simulink library "sm_wheel_loader_lib"  (R2025a)
settings: Solver=VariableStepAuto  StartTime=0.0  StopTime=10.0  RelTol=1e-3
undefined symbols (not defined in the file): AToTOrificeVector, BiPOrificeVector, boomHEArea, boomREArea, BToTOrificeVector, fluids, GRake, GToothL, GToothR, HMPST, HydFcnParams, logLoad, Position, PToAOrificeVector, PToBOrificeVector, RakeL, RakeR, testInput, Wheel_Loader, X, Y, Z
libraries: sm_lib x694, fl_lib x183, nesl_utility x74, SimscapeFluids_lib x62, sdl_lib x25, cvt_components_lib x25, simulink_extras x5, $bdroot x4, wheel_loader_contact_lib x4, ee_lib x2, SignalEditorBlockLib x1, batteryecm_lib x1
(part 20 of 26)

== system sm_wheel_loader_lib/Wheel Loader Vehicle/Driveline/Driveline/Driveline 1D/Planetary RL/Ring Gear ==
  Bolts : sm_lib/Body Elements/File Solid  ExtGeomFileName=InWheelPlanetary_Ring_Bolts.STEP  UnitType=FromFile  ExtGeomFileUnits=m  StepReaderType=HEX  ExportConvexHullGeometry=off  InertiaType=Custom  BasedOnType=DensityFromFile  Density=1000  DensityUnits=kg/m^3  Mass=Wheel_Loader.bodyGroups(74).subGroups(2).inertialProperties.mass  MassUnits=kg  CenterOfMass=Wheel_Loader.bodyGroups(74).subGroups(2).inertialProperties.centerOfMass  CenterOfMassUnits=m  MomentsOfInertia=Wheel_Loader.bodyGroups(74).subGroups(2).inertialProperties.momentsOfInertia  MomentsOfInertiaUnits=kg*m^2  ProductsOfInertia=Wheel_Loader.bodyGroups(74).subGroups(2).inertialProperties.productsOfInertia  ProductsOfInertiaUnits=kg*m^2  GraphicType=FromGeometry  MarkerShape=Sphere  MarkerSize=10  GraphicVisPropType=SimpleVisualProperties  GraphicDiffuseColor=Wheel_Loader.bodyGroups(74).subGroups(2).visualProperties.rgb  GraphicOpacity=Wheel_Loader.bodyGroups(74).subGroups(2).visualProperties.opacity  GraphicSpecularColor=[0.5 0.5 0.5 1.0]  GraphicAmbientColor=[0.15 0.15 0.15 1.0]  GraphicEmissiveColor=[0.0 0.0 0.0 1.0]  GraphicShininess=75  DoExposeReferenceFrame=on  SerializedFrames=<Frames/>
  Ring : sm_lib/Body Elements/File Solid  ExtGeomFileName=InWheelPlanetary_Ring.STEP  UnitType=FromFile  ExtGeomFileUnits=m  StepReaderType=HEX  ExportConvexHullGeometry=off  InertiaType=Custom  BasedOnType=DensityFromFile  Density=1000  DensityUnits=kg/m^3  Mass=Wheel_Loader.bodyGroups(74).subGroups(1).inertialProperties.mass  MassUnits=kg  CenterOfMass=Wheel_Loader.bodyGroups(74).subGroups(1).inertialProperties.centerOfMass  CenterOfMassUnits=m  MomentsOfInertia=Wheel_Loader.bodyGroups(74).subGroups(1).inertialProperties.momentsOfInertia  MomentsOfInertiaUnits=kg*m^2  ProductsOfInertia=Wheel_Loader.bodyGroups(74).subGroups(1).inertialProperties.productsOfInertia  ProductsOfInertiaUnits=kg*m^2  GraphicType=FromGeometry  MarkerShape=Sphere  MarkerSize=10  GraphicVisPropType=SimpleVisualProperties  GraphicDiffuseColor=Wheel_Loader.bodyGroups(74).subGroups(1).visualProperties.rgb  GraphicOpacity=Wheel_Loader.bodyGroups(74).subGroups(1).visualProperties.opacity  GraphicSpecularColor=[0.5 0.5 0.5 1.0]  GraphicAmbientColor=[0.15 0.15 0.15 1.0]  GraphicEmissiveColor=[0.0 0.0 0.0 1.0]  GraphicShininess=75  DoExposeReferenceFrame=on  SerializedFrames=<Frames/>
  RingGear_Center : sm_lib/Frames and Transforms/Rigid Transform  RotationMethod=RotationMatrix  FollAlignAxisA=+X  BaseAlignAxisA=+Y  FollAlignAxisB=+Y  BaseAlignAxisB=+Z  RotationStandardAxis=+Z  RotationAngle=0.0  RotationAngleUnits=deg  RotationArbitraryAxis=[0 0 1]  RotationSequenceAxes=FollowerAxes  RotationSequence=XYX  RotationSequenceAngles=[0 0 0]  RotationSequenceAnglesUnits=deg  RotationMatrix=Wheel_Loader.coordSys(58).transform.rotation  Quaternion=[1 0 0 0]  TranslationMethod=Cartesian  TranslationCartesianOffset=Wheel_Loader.coordSys(58).transform.translation  TranslationCartesianOffsetUnits=m  TranslationStandardAxis=+Z  TranslationStandardOffset=0  TranslationStandardOffsetUnits=m  TranslationROffset=0  TranslationROffsetUnits=m  TranslationThetaOffset=0  TranslationThetaOffsetUnits=deg  TranslationZOffset=0  TranslationZOffsetUnits=m
  B : PMIOPort  Side=Left
  connections:
  RingGear_Center/RConn1 -- B/RConn1
  Bolts/RConn1 -- RingGear_Center/LConn1 -- Ring/RConn1

== system sm_wheel_loader_lib/Wheel Loader Vehicle/Driveline/Driveline/Driveline 1D/Planetary RR/Carrier ==
  Bolts : sm_lib/Body Elements/File Solid  ExtGeomFileName=InWheelPlanetary_Carrier_Bolts.STEP  UnitType=FromFile  ExtGeomFileUnits=m  StepReaderType=HEX  ExportConvexHullGeometry=off  InertiaType=Custom  BasedOnType=DensityFromFile  Density=1000  DensityUnits=kg/m^3  Mass=Wheel_Loader.bodyGroups(75).subGroups(2).inertialProperties.mass  MassUnits=kg  CenterOfMass="Wheel_Loader.bodyGroups(75).subGroups(2).inertialProperties.centerOfMass-[0 0.000000601963208   0.000000302490290]'"  CenterOfMassUnits=m  MomentsOfInertia=Wheel_Loader.bodyGroups(75).subGroups(2).inertialProperties.momentsOfInertia  MomentsOfInertiaUnits=kg*m^2  ProductsOfInertia=Wheel_Loader.bodyGroups(75).subGroups(2).inertialProperties.productsOfInertia  ProductsOfInertiaUnits=kg*m^2  GraphicType=FromGeometry  MarkerShape=Sphere  MarkerSize=10  GraphicVisPropType=SimpleVisualProperties  GraphicDiffuseColor=Wheel_Loader.bodyGroups(75).subGroups(2).visualProperties.rgb  GraphicOpacity=casing_opc  GraphicSpecularColor=[0.5 0.5 0.5 1.0]  GraphicAmbientColor=[0.15 0.15 0.15 1.0]  GraphicEmissiveColor=[0.0 0.0 0.0 1.0]  GraphicShininess=75  DoExposeReferenceFrame=on  SerializedFrames=<Frames/>
  Carrier : sm_lib/Body Elements/File Solid  ExtGeomFileName=InWheelPlanetary_Carrier.STEP  UnitType=FromFile  ExtGeomFileUnits=m  StepReaderType=HEX  ExportConvexHullGeometry=off  InertiaType=Custom  BasedOnType=DensityFromFile  Density=1000  DensityUnits=kg/m^3  Mass=Wheel_Loader.bodyGroups(75).subGroups(1).inertialProperties.mass  MassUnits=kg  CenterOfMass="Wheel_Loader.bodyGroups(75).subGroups(1).inertialProperties.centerOfMass-[0 -0.000000000960056  -0.000000002279457]'"  CenterOfMassUnits=m  MomentsOfInertia=Wheel_Loader.bodyGroups(75).subGroups(1).inertialProperties.momentsOfInertia  MomentsOfInertiaUnits=kg*m^2  ProductsOfInertia=Wheel_Loader.bodyGroups(75).subGroups(1).inertialProperties.productsOfInertia  ProductsOfInertiaUnits=kg*m^2  GraphicType=FromGeometry  MarkerShape=Sphere  MarkerSize=10  GraphicVisPropType=SimpleVisualProperties  GraphicDiffuseColor=Wheel_Loader.bodyGroups(75).subGroups(1).visualProperties.rgb  GraphicOpacity=casing_opc  GraphicSpecularColor=[0.5 0.5 0.5 1.0]  GraphicAmbientColor=[0.15 0.15 0.15 1.0]  GraphicEmissiveColor=[0.0 0.0 0.0 1.0]  GraphicShininess=75  DoExposeReferenceFrame=on  SerializedFrames=<Frames/>
  RT1_Carrier_Planet1 : sm_lib/Frames and Transforms/Rigid Transform  RotationMethod=StandardAxis  FollAlignAxisA=+X  BaseAlignAxisA=+Y  FollAlignAxisB=+Y  BaseAlignAxisB=+Z  RotationStandardAxis=+Z  RotationAngle=3.5  RotationAngleUnits=deg  RotationArbitraryAxis=[0 0 1]  RotationSequenceAxes=FollowerAxes  RotationSequence=XYX  RotationSequenceAngles=[0 0 0]  RotationSequenceAnglesUnits=deg  RotationMatrix=Wheel_Loader.coordSys(58).transform.rotation  Quaternion=[1 0 0 0]  TranslationMethod=None  TranslationCartesianOffset=Wheel_Loader.coordSys(58).transform.translation  TranslationCartesianOffsetUnits=m  TranslationStandardAxis=+X  TranslationStandardOffset=-0.037861875000022  TranslationStandardOffsetUnits=m  TranslationROffset=0  TranslationROffsetUnits=m  TranslationThetaOffset=0  TranslationThetaOffsetUnits=deg  TranslationZOffset=0  TranslationZOffsetUnits=m
  RT1_Carrier_Planet2 : sm_lib/Frames and Transforms/Rigid Transform  RotationMethod=StandardAxis  FollAlignAxisA=+X  BaseAlignAxisA=+Y  FollAlignAxisB=+Y  BaseAlignAxisB=+Z  RotationStandardAxis=+Z  RotationAngle=3.5+120  RotationAngleUnits=deg  RotationArbitraryAxis=[0 0 1]  RotationSequenceAxes=FollowerAxes  RotationSequence=XYX  RotationSequenceAngles=[0 0 0]  RotationSequenceAnglesUnits=deg  RotationMatrix=Wheel_Loader.coordSys(58).transform.rotation  Quaternion=[1 0 0 0]  TranslationMethod=None  TranslationCartesianOffset=Wheel_Loader.coordSys(58).transform.translation  TranslationCartesianOffsetUnits=m  TranslationStandardAxis=+X  TranslationStandardOffset=-0.037861875000022  TranslationStandardOffsetUnits=m  TranslationROffset=0  TranslationROffsetUnits=m  TranslationThetaOffset=0  TranslationThetaOffsetUnits=deg  TranslationZOffset=0  TranslationZOffsetUnits=m
  RT1_Carrier_Planet3 : sm_lib/Frames and Transforms/Rigid Transform  RotationMethod=StandardAxis  FollAlignAxisA=+X  BaseAlignAxisA=+Y  FollAlignAxisB=+Y  BaseAlignAxisB=+Z  RotationStandardAxis=+Z  RotationAngle=3.5+240  RotationAngleUnits=deg  RotationArbitraryAxis=[0 0 1]  RotationSequenceAxes=FollowerAxes  RotationSequence=XYX  RotationSequenceAngles=[0 0 0]  RotationSequenceAnglesUnits=deg  RotationMatrix=Wheel_Loader.coordSys(58).transform.rotation  Quaternion=[1 0 0 0]  TranslationMethod=None  TranslationCartesianOffset=Wheel_Loader.coordSys(58).transform.translation  TranslationCartesianOffsetUnits=m  TranslationStandardAxis=+X  TranslationStandardOffset=-0.037861875000022  TranslationStandardOffsetUnits=m  TranslationROffset=0  TranslationROffsetUnits=m  TranslationThetaOffset=0  TranslationThetaOffsetUnits=deg  TranslationZOffset=0  TranslationZOffsetUnits=m
  RT2_Carrier_Planet1 : sm_lib/Frames and Transforms/Rigid Transform  RotationMethod=StandardAxis  FollAlignAxisA=+X  BaseAlignAxisA=+Y  FollAlignAxisB=+Y  BaseAlignAxisB=+Z  RotationStandardAxis=+Z  RotationAngle=-3.5  RotationAngleUnits=deg  RotationArbitraryAxis=[0 0 1]  RotationSequenceAxes=FollowerAxes  RotationSequence=XYX  RotationSequenceAngles=[0 0 0]  RotationSequenceAnglesUnits=deg  RotationMatrix=Wheel_Loader.coordSys(58).transform.rotation  Quaternion=[1 0 0 0]  TranslationMethod=StandardAxis  TranslationCartesianOffset=Wheel_Loader.coordSys(58).transform.translation  TranslationCartesianOffsetUnits=m  TranslationStandardAxis=+X  TranslationStandardOffset=-0.0378618750  TranslationStandardOffsetUnits=m  TranslationROffset=0  TranslationROffsetUnits=m  TranslationThetaOffset=0  TranslationThetaOffsetUnits=deg  TranslationZOffset=0  TranslationZOffsetUnits=m
  RT2_Carrier_Planet2 : sm_lib/Frames and Transforms/Rigid Transform  RotationMethod=StandardAxis  FollAlignAxisA=+X  BaseAlignAxisA=+Y  FollAlignAxisB=+Y  BaseAlignAxisB=+Z  RotationStandardAxis=+Z  RotationAngle=-3.5  RotationAngleUnits=deg  RotationArbitraryAxis=[0 0 1]  RotationSequenceAxes=FollowerAxes  RotationSequence=XYX  RotationSequenceAngles=[0 0 0]  RotationSequenceAnglesUnits=deg  RotationMatrix=Wheel_Loader.coordSys(58).transform.rotation  Quaternion=[1 0 0 0]  TranslationMethod=StandardAxis  TranslationCartesianOffset=Wheel_Loader.coordSys(58).transform.translation  TranslationCartesianOffsetUnits=m  TranslationStandardAxis=+X  TranslationStandardOffset=-0.0378618750  TranslationStandardOffsetUnits=m  TranslationROffset=0  TranslationROffsetUnits=m  TranslationThetaOffset=0  TranslationThetaOffsetUnits=deg  TranslationZOffset=0  TranslationZOffsetUnits=m
  RT2_Carrier_Planet3 : sm_lib/Frames and Transforms/Rigid Transform  RotationMethod=StandardAxis  FollAlignAxisA=+X  BaseAlignAxisA=+Y  FollAlignAxisB=+Y  BaseAlignAxisB=+Z  RotationStandardAxis=+Z  RotationAngle=-3.5  RotationAngleUnits=deg  RotationArbitraryAxis=[0 0 1]  RotationSequenceAxes=FollowerAxes  RotationSequence=XYX  RotationSequenceAngles=[0 0 0]  RotationSequenceAnglesUnits=deg  RotationMatrix=Wheel_Loader.coordSys(58).transform.rotation  Quaternion=[1 0 0 0]  TranslationMethod=StandardAxis  TranslationCartesianOffset=Wheel_Loader.coordSys(58).transform.translation  TranslationCartesianOffsetUnits=m  TranslationStandardAxis=+X  TranslationStandardOffset=-0.0378618750  TranslationStandardOffsetUnits=m  TranslationROffset=0  TranslationROffsetUnits=m  TranslationThetaOffset=0  TranslationThetaOffsetUnits=deg  TranslationZOffset=0  TranslationZOffsetUnits=m
  RT_RearAxle_Carrier : sm_lib/Frames and Transforms/Rigid Transform  RotationMethod=RotationMatrix  FollAlignAxisA=+X  BaseAlignAxisA=+Y  FollAlignAxisB=+Y  BaseAlignAxisB=+Z  RotationStandardAxis=+Z  RotationAngle=0.0  RotationAngleUnits=deg  RotationArbitraryAxis=[0 0 1]  RotationSequenceAxes=FollowerAxes  RotationSequence=XYX  RotationSequenceAngles=[0 0 0]  RotationSequenceAnglesUnits=deg  RotationMatrix=Wheel_Loader.coordSys(58).transform.rotation  Quaternion=[1 0 0 0]  TranslationMethod=Cartesian  TranslationCartesianOffset=Wheel_Loader.coordSys(58).transform.translation  TranslationCartesianOffsetUnits=m  TranslationStandardAxis=+Z  TranslationStandardOffset=0  TranslationStandardOffsetUnits=m  TranslationROffset=0  TranslationROffsetUnits=m  TranslationThetaOffset=0  TranslationThetaOffsetUnits=deg  TranslationZOffset=0  TranslationZOffsetUnits=m
  B : PMIOPort  Side=Left
  F1 : PMIOPort  Port=2  Side=Right
  F2 : PMIOPort  Port=3  Side=Right
  F3 : PMIOPort  Port=4  Side=Right
  connections:
  F3/RConn1 -- RT2_Carrier_Planet3/RConn1
  RT2_Carrier_Planet3/LConn1 -- RT1_Carrier_Planet3/RConn1
  RT2_Carrier_Planet2/LConn1 -- RT1_Carrier_Planet2/RConn1
  F2/RConn1 -- RT2_Carrier_Planet2/RConn1
  Carrier/RConn1 -- RT_RearAxle_Carrier/LConn1 -- Bolts/RConn1
  RT1_Carrier_Planet3/LConn1 -- RT1_Carrier_Planet2/LConn1 -- RT1_Carrier_Planet1/LConn1 -- RT_RearAxle_Carrier/RConn1 -- B/RConn1
  F1/RConn1 -- RT2_Carrier_Planet1/RConn1
  RT2_Carrier_Planet1/LConn1 -- RT1_Carrier_Planet1/RConn1

== system sm_wheel_loader_lib/Wheel Loader Vehicle/Driveline/Driveline/Driveline 1D/Planetary RR/Ring Gear ==
  Bolts : sm_lib/Body Elements/File Solid  ExtGeomFileName=InWheelPlanetary_Ring_Bolts.STEP  UnitType=FromFile  ExtGeomFileUnits=m  StepReaderType=HEX  ExportConvexHullGeometry=off  InertiaType=Custom  BasedOnType=DensityFromFile  Density=1000  DensityUnits=kg/m^3  Mass=Wheel_Loader.bodyGroups(74).subGroups(2).inertialProperties.mass  MassUnits=kg  CenterOfMass=Wheel_Loader.bodyGroups(74).subGroups(2).inertialProperties.centerOfMass  CenterOfMassUnits=m  MomentsOfInertia=Wheel_Loader.bodyGroups(74).subGroups(2).inertialProperties.momentsOfInertia  MomentsOfInertiaUnits=kg*m^2  ProductsOfInertia=Wheel_Loader.bodyGroups(74).subGroups(2).inertialProperties.productsOfInertia  ProductsOfInertiaUnits=kg*m^2  GraphicType=FromGeometry  MarkerShape=Sphere  MarkerSize=10  GraphicVisPropType=SimpleVisualProperties  GraphicDiffuseColor=Wheel_Loader.bodyGroups(74).subGroups(2).visualProperties.rgb  GraphicOpacity=Wheel_Loader.bodyGroups(74).subGroups(2).visualProperties.opacity  GraphicSpecularColor=[0.5 0.5 0.5 1.0]  GraphicAmbientColor=[0.15 0.15 0.15 1.0]  GraphicEmissiveColor=[0.0 0.0 0.0 1.0]  GraphicShininess=75  DoExposeReferenceFrame=on  SerializedFrames=<Frames/>
  Ring : sm_lib/Body Elements/File Solid  ExtGeomFileName=InWheelPlanetary_Ring.STEP  UnitType=FromFile  ExtGeomFileUnits=m  StepReaderType=HEX  ExportConvexHullGeometry=off  InertiaType=Custom  BasedOnType=DensityFromFile  Density=1000  DensityUnits=kg/m^3  Mass=Wheel_Loader.bodyGroups(74).subGroups(1).inertialProperties.mass  MassUnits=kg  CenterOfMass=Wheel_Loader.bodyGroups(74).subGroups(1).inertialProperties.centerOfMass  CenterOfMassUnits=m  MomentsOfInertia=Wheel_Loader.bodyGroups(74).subGroups(1).inertialProperties.momentsOfInertia  MomentsOfInertiaUnits=kg*m^2  ProductsOfInertia=Wheel_Loader.bodyGroups(74).subGroups(1).inertialProperties.productsOfInertia  ProductsOfInertiaUnits=kg*m^2  GraphicType=FromGeometry  MarkerShape=Sphere  MarkerSize=10  GraphicVisPropType=SimpleVisualProperties  GraphicDiffuseColor=Wheel_Loader.bodyGroups(74).subGroups(1).visualProperties.rgb  GraphicOpacity=Wheel_Loader.bodyGroups(74).subGroups(1).visualProperties.opacity  GraphicSpecularColor=[0.5 0.5 0.5 1.0]  GraphicAmbientColor=[0.15 0.15 0.15 1.0]  GraphicEmissiveColor=[0.0 0.0 0.0 1.0]  GraphicShininess=75  DoExposeReferenceFrame=on  SerializedFrames=<Frames/>
  RingGear_Center : sm_lib/Frames and Transforms/Rigid Transform  RotationMethod=RotationMatrix  FollAlignAxisA=+X  BaseAlignAxisA=+Y  FollAlignAxisB=+Y  BaseAlignAxisB=+Z  RotationStandardAxis=+Z  RotationAngle=0.0  RotationAngleUnits=deg  RotationArbitraryAxis=[0 0 1]  RotationSequenceAxes=FollowerAxes  RotationSequence=XYX  RotationSequenceAngles=[0 0 0]  RotationSequenceAnglesUnits=deg  RotationMatrix=Wheel_Loader.coordSys(58).transform.rotation  Quaternion=[1 0 0 0]  TranslationMethod=Cartesian  TranslationCartesianOffset=Wheel_Loader.coordSys(58).transform.translation  TranslationCartesianOffsetUnits=m  TranslationStandardAxis=+Z  TranslationStandardOffset=0  TranslationStandardOffsetUnits=m  TranslationROffset=0  TranslationROffsetUnits=m  TranslationThetaOffset=0  TranslationThetaOffsetUnits=deg  TranslationZOffset=0  TranslationZOffsetUnits=m
  B : PMIOPort  Side=Left
  connections:
  Ring/RConn1 -- RingGear_Center/LConn1 -- Bolts/RConn1
  RingGear_Center/RConn1 -- B/RConn1

== system sm_wheel_loader_lib/Wheel Loader Vehicle/Driveline/Driveline/Driveline 3D/Center Shaft/Center Bearing ==
  Center_Bearing : sm_lib/Body Elements/File Solid  ExtGeomFileName=Driveline_Center_Bearing.STEP  UnitType=FromFile  ExtGeomFileUnits=m  StepReaderType=HEX  ExportConvexHullGeometry=off  InertiaType=Custom  BasedOnType=DensityFromFile  Density=1000  DensityUnits=kg/m^3  Mass=Wheel_Loader.bodyGroups(41).subGroups(1).inertialProperties.mass  MassUnits=kg  CenterOfMass=Wheel_Loader.bodyGroups(41).subGroups(1).inertialProperties.centerOfMass  CenterOfMassUnits=m  MomentsOfInertia=Wheel_Loader.bodyGroups(41).subGroups(1).inertialProperties.momentsOfInertia  MomentsOfInertiaUnits=kg*m^2  ProductsOfInertia=Wheel_Loader.bodyGroups(41).subGroups(1).inertialProperties.productsOfInertia  ProductsOfInertiaUnits=kg*m^2  GraphicType=FromGeometry  MarkerShape=Sphere  MarkerSize=10  GraphicVisPropType=SimpleVisualProperties  GraphicDiffuseColor=Wheel_Loader.bodyGroups(41).subGroups(1).visualProperties.rgb  GraphicOpacity=Wheel_Loader.bodyGroups(41).subGroups(1).visualProperties.opacity  GraphicSpecularColor=[0.5 0.5 0.5 1.0]  GraphicAmbientColor=[0.15 0.15 0.15 1.0]  GraphicEmissiveColor=[0.0 0.0 0.0 1.0]  GraphicShininess=75  DoExposeReferenceFrame=on  SerializedFrames=<Frames/>
  RT_MidShipShaft_CentreBearingDriveShaft : sm_lib/Frames and Transforms/Rigid Transform  RotationMethod=RotationMatrix  FollAlignAxisA=+X  BaseAlignAxisA=+Y  FollAlignAxisB=+Y  BaseAlignAxisB=+Z  RotationStandardAxis=+Z  RotationAngle=0.0  RotationAngleUnits=deg  RotationArbitraryAxis=[0 0 1]  RotationSequenceAxes=FollowerAxes  RotationSequence=XYX  RotationSequenceAngles=[0 0 0]  RotationSequenceAnglesUnits=deg  RotationMatrix=Wheel_Loader.coordSys(22).transform.rotation  Quaternion=[1 0 0 0]  TranslationMethod=Cartesian  TranslationCartesianOffset=Wheel_Loader.coordSys(22).transform.translation  TranslationCartesianOffsetUnits=m  TranslationStandardAxis=+Z  TranslationStandardOffset=0  TranslationStandardOffsetUnits=m  TranslationROffset=0  TranslationROffsetUnits=m  TranslationThetaOffset=0  TranslationThetaOffsetUnits=deg  TranslationZOffset=0  TranslationZOffsetUnits=m
  RT_RearDriveShaft_CenterBearingDriveShaft : sm_lib/Frames and Transforms/Rigid Transform  RotationMethod=RotationMatrix  FollAlignAxisA=+X  BaseAlignAxisA=+Y  FollAlignAxisB=+Y  BaseAlignAxisB=+Z  RotationStandardAxis=+Z  RotationAngle=0.0  RotationAngleUnits=deg  RotationArbitraryAxis=[0 0 1]  RotationSequenceAxes=FollowerAxes  RotationSequence=XYX  RotationSequenceAngles=[0 0 0]  RotationSequenceAnglesUnits=deg  RotationMatrix=Wheel_Loader.coordSys(22).transform.rotation  Quaternion=[1 0 0 0]  TranslationMethod=Cartesian  TranslationCartesianOffset=Wheel_Loader.coordSys(22).transform.translation  TranslationCartesianOffsetUnits=m  TranslationStandardAxis=+Z  TranslationStandardOffset=0  TranslationStandardOffsetUnits=m  TranslationROffset=0  TranslationROffsetUnits=m  TranslationThetaOffset=0  TranslationThetaOffsetUnits=deg  TranslationZOffset=0  TranslationZOffsetUnits=m
  B1 : PMIOPort  Side=Left
  B2 : PMIOPort  Port=2  Side=Right
  connections:
  RT_RearDriveShaft_CenterBearingDriveShaft/RConn1 -- B2/RConn1
  RT_MidShipShaft_CentreBearingDriveShaft/RConn1 -- B1/RConn1
  Center_Bearing/RConn1 -- RT_MidShipShaft_CentreBearingDriveShaft/LConn1 -- RT_RearDriveShaft_CenterBearingDriveShaft/LConn1

== system sm_wheel_loader_lib/Wheel Loader Vehicle/Driveline/Driveline/Driveline 3D/Center Shaft/Shaft Midship ==
  Intermediate_Shaft_Midship : sm_lib/Body Elements/File Solid  ExtGeomFileName=Driveline_Intermediate_Shaft_Midship.STEP  UnitType=FromFile  ExtGeomFileUnits=m  StepReaderType=HEX  ExportConvexHullGeometry=off  InertiaType=Custom  BasedOnType=DensityFromFile  Density=1000  DensityUnits=kg/m^3  Mass=Wheel_Loader.bodyGroups(40).subGroups(1).inertialProperties.mass  MassUnits=kg  CenterOfMass=Wheel_Loader.bodyGroups(40).subGroups(1).inertialProperties.centerOfMass  CenterOfMassUnits=m  MomentsOfInertia=Wheel_Loader.bodyGroups(40).subGroups(1).inertialProperties.momentsOfInertia  MomentsOfInertiaUnits=kg*m^2  ProductsOfInertia=Wheel_Loader.bodyGroups(40).subGroups(1).inertialProperties.productsOfInertia  ProductsOfInertiaUnits=kg*m^2  GraphicType=FromGeometry  MarkerShape=Sphere  MarkerSize=10  GraphicVisPropType=SimpleVisualProperties  GraphicDiffuseColor=Wheel_Loader.bodyGroups(40).subGroups(1).visualProperties.rgb  GraphicOpacity=Wheel_Loader.bodyGroups(40).subGroups(1).visualProperties.opacity  GraphicSpecularColor=[0.5 0.5 0.5 1.0]  GraphicAmbientColor=[0.15 0.15 0.15 1.0]  GraphicEmissiveColor=[0.0 0.0 0.0 1.0]  GraphicShininess=75  DoExposeReferenceFrame=on  SerializedFrames=<Frames/>
  RT_FrontDriveShaft_MidShipShaft : sm_lib/Frames and Transforms/Rigid Transform  RotationMethod=RotationMatrix  FollAlignAxisA=+X  BaseAlignAxisA=+Y  FollAlignAxisB=+Y  BaseAlignAxisB=+Z  RotationStandardAxis=+Z  RotationAngle=0.0  RotationAngleUnits=deg  RotationArbitraryAxis=[0 0 1]  RotationSequenceAxes=FollowerAxes  RotationSequence=XYX  RotationSequenceAngles=[0 0 0]  RotationSequenceAnglesUnits=deg  RotationMatrix=Wheel_Loader.coordSys(22).transform.rotation  Quaternion=[1 0 0 0]  TranslationMethod=Cartesian  TranslationCartesianOffset=Wheel_Loader.coordSys(22).transform.translation  TranslationCartesianOffsetUnits=m  TranslationStandardAxis=+Z  TranslationStandardOffset=0  TranslationStandardOffsetUnits=m  TranslationROffset=0  TranslationROffsetUnits=m  TranslationThetaOffset=0  TranslationThetaOffsetUnits=deg  TranslationZOffset=0  TranslationZOffsetUnits=m
  B1 : PMIOPort  Side=Left
  F1 : PMIOPort  Port=2  Side=Right
  connections:
  F1/RConn1 -- RT_FrontDriveShaft_MidShipShaft/RConn1 -- B1/RConn1
  Intermediate_Shaft_Midship/RConn1 -- RT_FrontDriveShaft_MidShipShaft/LConn1

== system sm_wheel_loader_lib/Wheel Loader Vehicle/Driveline/Driveline/Driveline 3D/Differential F/Ring Gear ==
  Casing_A : sm_lib/Body Elements/File Solid  ExtGeomFileName=DiffF_Casing_A.STEP  UnitType=FromFile  ExtGeomFileUnits=m  StepReaderType=HEX  ExportConvexHullGeometry=off  InertiaType=Custom  BasedOnType=DensityFromFile  Density=1000  DensityUnits=kg/m^3  Mass=Wheel_Loader.bodyGroups(68).subGroups(1).inertialProperties.mass  MassUnits=kg  CenterOfMass=Wheel_Loader.bodyGroups(68).subGroups(1).inertialProperties.centerOfMass  CenterOfMassUnits=m  MomentsOfInertia=Wheel_Loader.bodyGroups(68).subGroups(1).inertialProperties.momentsOfInertia  MomentsOfInertiaUnits=kg*m^2  ProductsOfInertia=Wheel_Loader.bodyGroups(68).subGroups(1).inertialProperties.productsOfInertia  ProductsOfInertiaUnits=kg*m^2  GraphicType=FromGeometry  MarkerShape=Sphere  MarkerSize=10  GraphicVisPropType=SimpleVisualProperties  GraphicDiffuseColor=Wheel_Loader.bodyGroups(68).subGroups(1).visualProperties.rgb  GraphicOpacity=diff_casing_opc  GraphicSpecularColor=[0.5 0.5 0.5 1.0]  GraphicAmbientColor=[0.15 0.15 0.15 1.0]  GraphicEmissiveColor=[0.0 0.0 0.0 1.0]  GraphicShininess=75  DoExposeReferenceFrame=on  SerializedFrames=<Frames/>
  Casing_B : sm_lib/Body Elements/File Solid  ExtGeomFileName=DiffF_Casing_B.STEP  UnitType=FromFile  ExtGeomFileUnits=m  StepReaderType=HEX  ExportConvexHullGeometry=off  InertiaType=Custom  BasedOnType=DensityFromFile  Density=1000  DensityUnits=kg/m^3  Mass=Wheel_Loader.bodyGroups(68).subGroups(2).inertialProperties.mass  MassUnits=kg  CenterOfMass=Wheel_Loader.bodyGroups(68).subGroups(2).inertialProperties.centerOfMass  CenterOfMassUnits=m  MomentsOfInertia=Wheel_Loader.bodyGroups(68).subGroups(2).inertialProperties.momentsOfInertia  MomentsOfInertiaUnits=kg*m^2  ProductsOfInertia=Wheel_Loader.bodyGroups(68).subGroups(2).inertialProperties.productsOfInertia  ProductsOfInertiaUnits=kg*m^2  GraphicType=FromGeometry  MarkerShape=Sphere  MarkerSize=10  GraphicVisPropType=SimpleVisualProperties  GraphicDiffuseColor=Wheel_Loader.bodyGroups(68).subGroups(2).visualProperties.rgb  GraphicOpacity=diff_casing_opc  GraphicSpecularColor=[0.5 0.5 0.5 1.0]  GraphicAmbientColor=[0.15 0.15 0.15 1.0]  GraphicEmissiveColor=[0.0 0.0 0.0 1.0]  GraphicShininess=75  DoExposeReferenceFrame=on  SerializedFrames=<Frames/>
  RT_FDL_StubShaft_RingGear : sm_lib/Frames and Transforms/Rigid Transform  RotationMethod=RotationMatrix  FollAlignAxisA=+X  BaseAlignAxisA=+Y  FollAlignAxisB=+Y  BaseAlignAxisB=+Z  RotationStandardAxis=+Z  RotationAngle=0.0  RotationAngleUnits=deg  RotationArbitraryAxis=[0 0 1]  RotationSequenceAxes=FollowerAxes  RotationSequence=XYX  RotationSequenceAngles=[0 0 0]  RotationSequenceAnglesUnits=deg  RotationMatrix=Wheel_Loader.coordSys(43).transform.rotation  Quaternion=[1 0 0 0]  TranslationMethod=Cartesian  TranslationCartesianOffset=Wheel_Loader.coordSys(43).transform.translation  TranslationCartesianOffsetUnits=m  TranslationStandardAxis=+Z  TranslationStandardOffset=0  TranslationStandardOffsetUnits=m  TranslationROffset=0  TranslationROffsetUnits=m  TranslationThetaOffset=0  TranslationThetaOffsetUnits=deg  TranslationZOffset=0  TranslationZOffsetUnits=m
  RT_FDL_StubShaft_SideGear : sm_lib/Frames and Transforms/Rigid Transform  RotationMethod=RotationMatrix  FollAlignAxisA=+X  BaseAlignAxisA=+Y  FollAlignAxisB=+Y  BaseAlignAxisB=+Z  RotationStandardAxis=+Z  RotationAngle=0.0  RotationAngleUnits=deg  RotationArbitraryAxis=[0 0 1]  RotationSequenceAxes=FollowerAxes  RotationSequence=XYX  RotationSequenceAngles=[0 0 0]  RotationSequenceAnglesUnits=deg  RotationMatrix=Wheel_Loader.coordSys(51).transform.rotation  Quaternion=[1 0 0 0]  TranslationMethod=Cartesian  TranslationCartesianOffset=Wheel_Loader.coordSys(51).transform.translation  TranslationCartesianOffsetUnits=m  TranslationStandardAxis=+Z  TranslationStandardOffset=0  TranslationStandardOffsetUnits=m  TranslationROffset=0  TranslationROffsetUnits=m  TranslationThetaOffset=0  TranslationThetaOffsetUnits=deg  TranslationZOffset=0  TranslationZOffsetUnits=m
  Rigid Transform : sm_lib/Frames and Transforms/Rigid Transform  RotationMethod=None  FollAlignAxisA=+X  BaseAlignAxisA=+Y  FollAlignAxisB=+Y  BaseAlignAxisB=+Z  RotationStandardAxis=+Z  RotationAngle=0.0  RotationAngleUnits=deg  RotationArbitraryAxis=[0 0 1]  RotationSequenceAxes=FollowerAxes  RotationSequence=XYX  RotationSequenceAngles=[0 0 0]  RotationSequenceAnglesUnits=deg  RotationMatrix=[1 0 0; 0 1 0; 0 0 1]  Quaternion=[1 0 0 0]  TranslationMethod=Cartesian  TranslationCartesianOffset=-[0 -0.000000025687926 -0.000000034543427]  TranslationCartesianOffsetUnits=m  TranslationStandardAxis=+Z  TranslationStandardOffset=0  TranslationStandardOffsetUnits=m  TranslationROffset=0  TranslationROffsetUnits=m  TranslationThetaOffset=0  TranslationThetaOffsetUnits=deg  TranslationZOffset=0  TranslationZOffsetUnits=m
  Ring : sm_lib/Body Elements/File Solid  ExtGeomFileName=DiffF_Ring_Gear.STEP  UnitType=FromFile  ExtGeomFileUnits=m  StepReaderType=HEX  ExportConvexHullGeometry=off  InertiaType=Custom  BasedOnType=DensityFromFile  Density=1000  DensityUnits=kg/m^3  Mass=Wheel_Loader.bodyGroups(64).subGroups(1).inertialProperties.mass  MassUnits=kg  CenterOfMass=Wheel_Loader.bodyGroups(64).subGroups(1).inertialProperties.centerOfMass  CenterOfMassUnits=m  MomentsOfInertia=Wheel_Loader.bodyGroups(64).subGroups(1).inertialProperties.momentsOfInertia  MomentsOfInertiaUnits=kg*m^2  ProductsOfInertia=Wheel_Loader.bodyGroups(64).subGroups(1).inertialProperties.productsOfInertia  ProductsOfInertiaUnits=kg*m^2  GraphicType=FromGeometry  MarkerShape=Sphere  MarkerSize=10  GraphicVisPropType=SimpleVisualProperties  GraphicDiffuseColor=Wheel_Loader.bodyGroups(64).subGroups(1).visualProperties.rgb  GraphicOpacity=Wheel_Loader.bodyGroups(64).subGroups(1).visualProperties.opacity  GraphicSpecularColor=[0.5 0.5 0.5 1.0]  GraphicAmbientColor=[0.15 0.15 0.15 1.0]  GraphicEmissiveColor=[0.0 0.0 0.0 1.0]  GraphicShininess=75  DoExposeReferenceFrame=on  SerializedFrames=<Frames/>
  F : PMIOPort  Side=Right
  B : PMIOPort  Port=2  Side=Left
  connections:
  RT_FDL_StubShaft_SideGear/RConn1 -- F/RConn1
  B/RConn1 -- RT_FDL_StubShaft_RingGear/RConn1
  Casing_B/RConn1 -- Casing_A/RConn1 -- Rigid Transform/RConn1
  Rigid Transform/LConn1 -- RT_FDL_StubShaft_SideGear/LConn1 -- RT_FDL_StubShaft_RingGear/LConn1 -- Ring/RConn1

== system sm_wheel_loader_lib/Wheel Loader Vehicle/Driveline/Driveline/Driveline 3D/Differential F/Side Gear L ==
  RT_FDL_StubShaft_SideGear : sm_lib/Frames and Transforms/Rigid Transform  RotationMethod=RotationMatrix  FollAlignAxisA=+X  BaseAlignAxisA=+Y  FollAlignAxisB=+Y  BaseAlignAxisB=+Z  RotationStandardAxis=+Z  RotationAngle=0.0  RotationAngleUnits=deg  RotationArbitraryAxis=[0 0 1]  RotationSequenceAxes=FollowerAxes  RotationSequence=XYX  RotationSequenceAngles=[0 0 0]  RotationSequenceAnglesUnits=deg  RotationMatrix=Wheel_Loader.coordSys(51).transform.rotation  Quaternion=[1 0 0 0]  TranslationMethod=Cartesian  TranslationCartesianOffset=Wheel_Loader.coordSys(51).transform.translation  TranslationCartesianOffsetUnits=m  TranslationStandardAxis=+Z  TranslationStandardOffset=0  TranslationStandardOffsetUnits=m  TranslationROffset=0  TranslationROffsetUnits=m  TranslationThetaOffset=0  TranslationThetaOffsetUnits=deg  TranslationZOffset=0  TranslationZOffsetUnits=m
  Side_Gear_L : sm_lib/Body Elements/File Solid  ExtGeomFileName=DiffF_Side_Gear_L.STEP  UnitType=FromFile  ExtGeomFileUnits=m  StepReaderType=HEX  ExportConvexHullGeometry=off  InertiaType=Custom  BasedOnType=DensityFromFile  Density=1000  DensityUnits=kg/m^3  Mass=Wheel_Loader.bodyGroups(59).subGroups(1).inertialProperties.mass  MassUnits=kg  CenterOfMass=Wheel_Loader.bodyGroups(59).subGroups(1).inertialProperties.centerOfMass  CenterOfMassUnits=m  MomentsOfInertia=Wheel_Loader.bodyGroups(59).subGroups(1).inertialProperties.momentsOfInertia  MomentsOfInertiaUnits=kg*m^2  ProductsOfInertia=Wheel_Loader.bodyGroups(59).subGroups(1).inertialProperties.productsOfInertia  ProductsOfInertiaUnits=kg*m^2  GraphicType=FromGeometry  MarkerShape=Sphere  MarkerSize=10  GraphicVisPropType=SimpleVisualProperties  GraphicDiffuseColor=Wheel_Loader.bodyGroups(59).subGroups(1).visualProperties.rgb  GraphicOpacity=Wheel_Loader.bodyGroups(59).subGroups(1).visualProperties.opacity  GraphicSpecularColor=[0.5 0.5 0.5 1.0]  GraphicAmbientColor=[0.15 0.15 0.15 1.0]  GraphicEmissiveColor=[0.0 0.0 0.0 1.0]  GraphicShininess=75  DoExposeReferenceFrame=on  SerializedFrames=<Frames/>
  B : PMIOPort  Side=Left
  F : PMIOPort  Port=2  Side=Right
  connections:
  B/RConn1 -- F/RConn1 -- RT_FDL_StubShaft_SideGear/RConn1
  Side_Gear_L/RConn1 -- RT_FDL_StubShaft_SideGear/LConn1

== system sm_wheel_loader_lib/Wheel Loader Vehicle/Driveline/Driveline/Driveline 3D/Differential F/Side Gear R ==
  RT_FDSpiderGear2_FDRSideGear_BGC : sm_lib/Frames and Transforms/Rigid Transform  RotationMethod=RotationMatrix  FollAlignAxisA=+X  BaseAlignAxisA=+Y  FollAlignAxisB=+Y  BaseAlignAxisB=+Z  RotationStandardAxis=+Z  RotationAngle=0.0  RotationAngleUnits=deg  RotationArbitraryAxis=[0 0 1]  RotationSequenceAxes=FollowerAxes  RotationSequence=XYX  RotationSequenceAngles=[0 0 0]  RotationSequenceAnglesUnits=deg  RotationMatrix=Wheel_Loader.coordSys(49).transform.rotation  Quaternion=[1 0 0 0]  TranslationMethod=Cartesian  TranslationCartesianOffset=Wheel_Loader.coordSys(49).transform.translation  TranslationCartesianOffsetUnits=m  TranslationStandardAxis=+Z  TranslationStandardOffset=0  TranslationStandardOffsetUnits=m  TranslationROffset=0  TranslationROffsetUnits=m  TranslationThetaOffset=0  TranslationThetaOffsetUnits=deg  TranslationZOffset=0  TranslationZOffsetUnits=m
  Side_Gear_R : sm_lib/Body Elements/File Solid  ExtGeomFileName=DiffF_Side_Gear_R.STEP  UnitType=FromFile  ExtGeomFileUnits=m  StepReaderType=HEX  ExportConvexHullGeometry=off  InertiaType=Custom  BasedOnType=DensityFromFile  Density=1000  DensityUnits=kg/m^3  Mass=Wheel_Loader.bodyGroups(58).subGroups(1).inertialProperties.mass  MassUnits=kg  CenterOfMass=Wheel_Loader.bodyGroups(58).subGroups(1).inertialProperties.centerOfMass  CenterOfMassUnits=m  MomentsOfInertia=Wheel_Loader.bodyGroups(58).subGroups(1).inertialProperties.momentsOfInertia  MomentsOfInertiaUnits=kg*m^2  ProductsOfInertia=Wheel_Loader.bodyGroups(58).subGroups(1).inertialProperties.productsOfInertia  ProductsOfInertiaUnits=kg*m^2  GraphicType=FromGeometry  MarkerShape=Sphere  MarkerSize=10  GraphicVisPropType=SimpleVisualProperties  GraphicDiffuseColor=Wheel_Loader.bodyGroups(58).subGroups(1).visualProperties.rgb  GraphicOpacity=Wheel_Loader.bodyGroups(58).subGroups(1).visualProperties.opacity  GraphicSpecularColor=[0.5 0.5 0.5 1.0]  GraphicAmbientColor=[0.15 0.15 0.15 1.0]  GraphicEmissiveColor=[0.0 0.0 0.0 1.0]  GraphicShininess=75  DoExposeReferenceFrame=on  SerializedFrames=<Frames/>
  B : PMIOPort  Side=Left
  F : PMIOPort  Port=2  Side=Right
  connections:
  B/RConn1 -- RT_FDSpiderGear2_FDRSideGear_BGC/RConn1 -- F/RConn1
  Side_Gear_R/RConn1 -- RT_FDSpiderGear2_FDRSideGear_BGC/LConn1

== system sm_wheel_loader_lib/Wheel Loader Vehicle/Driveline/Driveline/Driveline 3D/Differential F/Spider Gear 1 ==
  Gear : sm_lib/Body Elements/File Solid  ExtGeomFileName=DiffF_Spider_Gear1.STEP  UnitType=FromFile  ExtGeomFileUnits=m  StepReaderType=HEX  ExportConvexHullGeometry=off  InertiaType=Custom  BasedOnType=DensityFromFile  Density=1000  DensityUnits=kg/m^3  Mass=Wheel_Loader.bodyGroups(60).subGroups(1).inertialProperties.mass  MassUnits=kg  CenterOfMass=Wheel_Loader.bodyGroups(60).subGroups(1).inertialProperties.centerOfMass  CenterOfMassUnits=m  MomentsOfInertia=Wheel_Loader.bodyGroups(60).subGroups(1).inertialProperties.momentsOfInertia  MomentsOfInertiaUnits=kg*m^2  ProductsOfInertia=Wheel_Loader.bodyGroups(60).subGroups(1).inertialProperties.productsOfInertia  ProductsOfInertiaUnits=kg*m^2  GraphicType=FromGeometry  MarkerShape=Sphere  MarkerSize=10  GraphicVisPropType=SimpleVisualProperties  GraphicDiffuseColor=Wheel_Loader.bodyGroups(60).subGroups(1).visualProperties.rgb  GraphicOpacity=Wheel_Loader.bodyGroups(60).subGroups(1).visualProperties.opacity  GraphicSpecularColor=[0.5 0.5 0.5 1.0]  GraphicAmbientColor=[0.15 0.15 0.15 1.0]  GraphicEmissiveColor=[0.0 0.0 0.0 1.0]  GraphicShininess=75  DoExposeReferenceFrame=on  SerializedFrames=<Frames/>
  RT_FD_Casing_SpiderGear4 : sm_lib/Frames and Transforms/Rigid Transform  RotationMethod=RotationMatrix  FollAlignAxisA=+X  BaseAlignAxisA=+Y  FollAlignAxisB=+Y  BaseAlignAxisB=+Z  RotationStandardAxis=+Z  RotationAngle=0.0  RotationAngleUnits=deg  RotationArbitraryAxis=[0 0 1]  RotationSequenceAxes=FollowerAxes  RotationSequence=XYX  RotationSequenceAngles=[0 0 0]  RotationSequenceAnglesUnits=deg  RotationMatrix=Wheel_Loader.coordSys(45).transform.rotation  Quaternion=[1 0 0 0]  TranslationMethod=Cartesian  TranslationCartesianOffset=Wheel_Loader.coordSys(45).transform.translation  TranslationCartesianOffsetUnits=m  TranslationStandardAxis=+Z  TranslationStandardOffset=0  TranslationStandardOffsetUnits=m  TranslationROffset=0  TranslationROffsetUnits=m  TranslationThetaOffset=0  TranslationThetaOffsetUnits=deg  TranslationZOffset=0  TranslationZOffsetUnits=m
  Shaft : sm_lib/Body Elements/File Solid  ExtGeomFileName=DiffF_Spider_Gear1_Shaft.STEP  UnitType=FromFile  ExtGeomFileUnits=m  StepReaderType=HEX  ExportConvexHullGeometry=off  InertiaType=Custom  BasedOnType=DensityFromFile  Density=1000  DensityUnits=kg/m^3  Mass=Wheel_Loader.bodyGroups(60).subGroups(2).inertialProperties.mass  MassUnits=kg  CenterOfMass=Wheel_Loader.bodyGroups(60).subGroups(2).inertialProperties.centerOfMass  CenterOfMassUnits=m  MomentsOfInertia=Wheel_Loader.bodyGroups(60).subGroups(2).inertialProperties.momentsOfInertia  MomentsOfInertiaUnits=kg*m^2  ProductsOfInertia=Wheel_Loader.bodyGroups(60).subGroups(2).inertialProperties.productsOfInertia  ProductsOfInertiaUnits=kg*m^2  GraphicType=FromGeometry  MarkerShape=Sphere  MarkerSize=10  GraphicVisPropType=SimpleVisualProperties  GraphicDiffuseColor=Wheel_Loader.bodyGroups(60).subGroups(2).visualProperties.rgb  GraphicOpacity=Wheel_Loader.bodyGroups(60).subGroups(2).visualProperties.opacity  GraphicSpecularColor=[0.5 0.5 0.5 1.0]  GraphicAmbientColor=[0.15 0.15 0.15 1.0]  GraphicEmissiveColor=[0.0 0.0 0.0 1.0]  GraphicShininess=75  DoExposeReferenceFrame=on  SerializedFrames=<Frames/>
  B : PMIOPort  Side=Left
  F : PMIOPort  Port=2  Side=Right
  connections:
  Gear/RConn1 -- Shaft/RConn1 -- RT_FD_Casing_SpiderGear4/LConn1
  B/RConn1 -- RT_FD_Casing_SpiderGear4/RConn1 -- F/RConn1

== system sm_wheel_loader_lib/Wheel Loader Vehicle/Driveline/Driveline/Driveline 3D/Differential F/Spider Gear 2 ==
  Gear : sm_lib/Body Elements/File Solid  ExtGeomFileName=DiffF_Spider_Gear2.STEP  UnitType=FromFile  ExtGeomFileUnits=m  StepReaderType=HEX  ExportConvexHullGeometry=off  InertiaType=Custom  BasedOnType=DensityFromFile  Density=1000  DensityUnits=kg/m^3  Mass=Wheel_Loader.bodyGroups(66).subGroups(1).inertialProperties.mass  MassUnits=kg  CenterOfMass=Wheel_Loader.bodyGroups(66).subGroups(1).inertialProperties.centerOfMass  CenterOfMassUnits=m  MomentsOfInertia=Wheel_Loader.bodyGroups(66).subGroups(1).inertialProperties.momentsOfInertia  MomentsOfInertiaUnits=kg*m^2  ProductsOfInertia=Wheel_Loader.bodyGroups(66).subGroups(1).inertialProperties.productsOfInertia  ProductsOfInertiaUnits=kg*m^2  GraphicType=FromGeometry  MarkerShape=Sphere  MarkerSize=10  GraphicVisPropType=SimpleVisualProperties  GraphicDiffuseColor=Wheel_Loader.bodyGroups(66).subGroups(1).visualProperties.rgb  GraphicOpacity=Wheel_Loader.bodyGroups(66).subGroups(1).visualProperties.opacity  GraphicSpecularColor=[0.5 0.5 0.5 1.0]  GraphicAmbientColor=[0.15 0.15 0.15 1.0]  GraphicEmissiveColor=[0.0 0.0 0.0 1.0]  GraphicShininess=75  DoExposeReferenceFrame=on  SerializedFrames=<Frames/>
  RT_FD_Casing_SpiderGear3 : sm_lib/Frames and Transforms/Rigid Transform  RotationMethod=RotationMatrix  FollAlignAxisA=+X  BaseAlignAxisA=+Y  FollAlignAxisB=+Y  BaseAlignAxisB=+Z  RotationStandardAxis=+Z  RotationAngle=0.0  RotationAngleUnits=deg  RotationArbitraryAxis=[0 0 1]  RotationSequenceAxes=FollowerAxes  RotationSequence=XYX  RotationSequenceAngles=[0 0 0]  RotationSequenceAnglesUnits=deg  RotationMatrix=Wheel_Loader.coordSys(53).transform.rotation  Quaternion=[1 0 0 0]  TranslationMethod=Cartesian  TranslationCartesianOffset=Wheel_Loader.coordSys(53).transform.translation  TranslationCartesianOffsetUnits=m  TranslationStandardAxis=+Z  TranslationStandardOffset=0  TranslationStandardOffsetUnits=m  TranslationROffset=0  TranslationROffsetUnits=m  TranslationThetaOffset=0  TranslationThetaOffsetUnits=deg  TranslationZOffset=0  TranslationZOffsetUnits=m
  Shaft : sm_lib/Body Elements/File Solid  ExtGeomFileName=DiffF_Spider_Gear2_Shaft.STEP  UnitType=FromFile  ExtGeomFileUnits=m  StepReaderType=HEX  ExportConvexHullGeometry=off  InertiaType=Custom  BasedOnType=DensityFromFile  Density=1000  DensityUnits=kg/m^3  Mass=Wheel_Loader.bodyGroups(66).subGroups(2).inertialProperties.mass  MassUnits=kg  CenterOfMass=Wheel_Loader.bodyGroups(66).subGroups(2).inertialProperties.centerOfMass  CenterOfMassUnits=m  MomentsOfInertia=Wheel_Loader.bodyGroups(66).subGroups(2).inertialProperties.momentsOfInertia  MomentsOfInertiaUnits=kg*m^2  ProductsOfInertia=Wheel_Loader.bodyGroups(66).subGroups(2).inertialProperties.productsOfInertia  ProductsOfInertiaUnits=kg*m^2  GraphicType=FromGeometry  MarkerShape=Sphere  MarkerSize=10  GraphicVisPropType=SimpleVisualProperties  GraphicDiffuseColor=Wheel_Loader.bodyGroups(66).subGroups(2).visualProperties.rgb  GraphicOpacity=Wheel_Loader.bodyGroups(66).subGroups(2).visualProperties.opacity  GraphicSpecularColor=[0.5 0.5 0.5 1.0]  GraphicAmbientColor=[0.15 0.15 0.15 1.0]  GraphicEmissiveColor=[0.0 0.0 0.0 1.0]  GraphicShininess=75  DoExposeReferenceFrame=on  SerializedFrames=<Frames/>
  B : PMIOPort  Side=Left
  F : PMIOPort  Port=2  Side=Right
  connections:
  RT_FD_Casing_SpiderGear3/RConn1 -- B/RConn1 -- F/RConn1
  RT_FD_Casing_SpiderGear3/LConn1 -- Gear/RConn1 -- Shaft/RConn1

== system sm_wheel_loader_lib/Wheel Loader Vehicle/Driveline/Driveline/Driveline 3D/Differential F/Stub Shaft L ==
  RT_FDLStubShaft_LFFDSunGear_Weld : sm_lib/Frames and Transforms/Rigid Transform  RotationMethod=RotationMatrix  FollAlignAxisA=+X  BaseAlignAxisA=+Y  FollAlignAxisB=+Y  BaseAlignAxisB=+Z  RotationStandardAxis=+Z  RotationAngle=0.0  RotationAngleUnits=deg  RotationArbitraryAxis=[0 0 1]  RotationSequenceAxes=FollowerAxes  RotationSequence=XYX  RotationSequenceAngles=[0 0 0]  RotationSequenceAnglesUnits=deg  RotationMatrix=Wheel_Loader.coordSys(70).transform.rotation  Quaternion=[1 0 0 0]  TranslationMethod=Cartesian  TranslationCartesianOffset=Wheel_Loader.coordSys(70).transform.translation  TranslationCartesianOffsetUnits=m  TranslationStandardAxis=+Z  TranslationStandardOffset=0  TranslationStandardOffsetUnits=m  TranslationROffset=0  TranslationROffsetUnits=m  TranslationThetaOffset=0  TranslationThetaOffsetUnits=deg  TranslationZOffset=0  TranslationZOffsetUnits=m
  RT_FDL_StubShaft_SideGear : sm_lib/Frames and Transforms/Rigid Transform  RotationMethod=RotationMatrix  FollAlignAxisA=+X  BaseAlignAxisA=+Y  FollAlignAxisB=+Y  BaseAlignAxisB=+Z  RotationStandardAxis=+Z  RotationAngle=0.0  RotationAngleUnits=deg  RotationArbitraryAxis=[0 0 1]  RotationSequenceAxes=FollowerAxes  RotationSequence=XYX  RotationSequenceAngles=[0 0 0]  RotationSequenceAnglesUnits=deg  RotationMatrix=Wheel_Loader.coordSys(51).transform.rotation  Quaternion=[1 0 0 0]  TranslationMethod=Cartesian  TranslationCartesianOffset=Wheel_Loader.coordSys(51).transform.translation  TranslationCartesianOffsetUnits=m  TranslationStandardAxis=+Z  TranslationStandardOffset=0  TranslationStandardOffsetUnits=m  TranslationROffset=0  TranslationROffsetUnits=m  TranslationThetaOffset=0  TranslationThetaOffsetUnits=deg  TranslationZOffset=0  TranslationZOffsetUnits=m
  Shaft : sm_lib/Body Elements/File Solid  ExtGeomFileName=DiffF_Stub_Shaft_L.STEP  UnitType=FromFile  ExtGeomFileUnits=m  StepReaderType=HEX  ExportConvexHullGeometry=off  InertiaType=Custom  BasedOnType=DensityFromFile  Density=1000  DensityUnits=kg/m^3  Mass=Wheel_Loader.bodyGroups(42).subGroups(1).inertialProperties.mass  MassUnits=kg  CenterOfMass=Wheel_Loader.bodyGroups(42).subGroups(1).inertialProperties.centerOfMass  CenterOfMassUnits=m  MomentsOfInertia=Wheel_Loader.bodyGroups(42).subGroups(1).inertialProperties.momentsOfInertia  MomentsOfInertiaUnits=kg*m^2  ProductsOfInertia=Wheel_Loader.bodyGroups(42).subGroups(1).inertialProperties.productsOfInertia  ProductsOfInertiaUnits=kg*m^2  GraphicType=FromGeometry  MarkerShape=Sphere  MarkerSize=10  GraphicVisPropType=SimpleVisualProperties  GraphicDiffuseColor=Wheel_Loader.bodyGroups(42).subGroups(1).visualProperties.rgb  GraphicOpacity=Wheel_Loader.bodyGroups(42).subGroups(1).visualProperties.opacity  GraphicSpecularColor=[0.5 0.5 0.5 1.0]  GraphicAmbientColor=[0.15 0.15 0.15 1.0]  GraphicEmissiveColor=[0.0 0.0 0.0 1.0]  GraphicShininess=75  DoExposeReferenceFrame=on  SerializedFrames=<Frames/>
  Spacer : sm_lib/Body Elements/File Solid  ExtGeomFileName=DiffF_Stub_Shaft_L_Spacer.STEP  UnitType=FromFile  ExtGeomFileUnits=m  StepReaderType=HEX  ExportConvexHullGeometry=off  InertiaType=Custom  BasedOnType=DensityFromFile  Density=1000  DensityUnits=kg/m^3  Mass=Wheel_Loader.bodyGroups(42).subGroups(2).inertialProperties.mass  MassUnits=kg  CenterOfMass=Wheel_Loader.bodyGroups(42).subGroups(2).inertialProperties.centerOfMass  CenterOfMassUnits=m  MomentsOfInertia=Wheel_Loader.bodyGroups(42).subGroups(2).inertialProperties.momentsOfInertia  MomentsOfInertiaUnits=kg*m^2  ProductsOfInertia=Wheel_Loader.bodyGroups(42).subGroups(2).inertialProperties.productsOfInertia  ProductsOfInertiaUnits=kg*m^2  GraphicType=FromGeometry  MarkerShape=Sphere  MarkerSize=10  GraphicVisPropType=SimpleVisualProperties  GraphicDiffuseColor=Wheel_Loader.bodyGroups(42).subGroups(2).visualProperties.rgb  GraphicOpacity=Wheel_Loader.bodyGroups(42).subGroups(2).visualProperties.opacity  GraphicSpecularColor=[0.5 0.5 0.5 1.0]  GraphicAmbientColor=[0.15 0.15 0.15 1.0]  GraphicEmissiveColor=[0.0 0.0 0.0 1.0]  GraphicShininess=75  DoExposeReferenceFrame=on  SerializedFrames=<Frames/>
  F3 : PMIOPort  Side=Left
  F1 : PMIOPort  Port=2  Side=Right
  connections:
  RT_FDLStubShaft_LFFDSunGear_Weld/RConn1 -- F3/RConn1
  RT_FDL_StubShaft_SideGear/RConn1 -- F1/RConn1
  RT_FDLStubShaft_LFFDSunGear_Weld/LConn1 -- RT_FDL_StubShaft_SideGear/LConn1 -- Shaft/RConn1 -- Spacer/RConn1
